simulink library "lib_IC_GFL"  (R2026a)
settings: Solver=VariableStepAuto
undefined symbols (not defined in the file): block_buses, block_DC_buses, block_DC_toM, block_idx, block_toM, buses_lf, DC, dparams, fref, invL, iTf, op_intconv_GFL, vdc_idx
libraries: sl_discontinuities x2, simulink x1
settings Model: Creator=atomas  LastModifiedBy=atomas

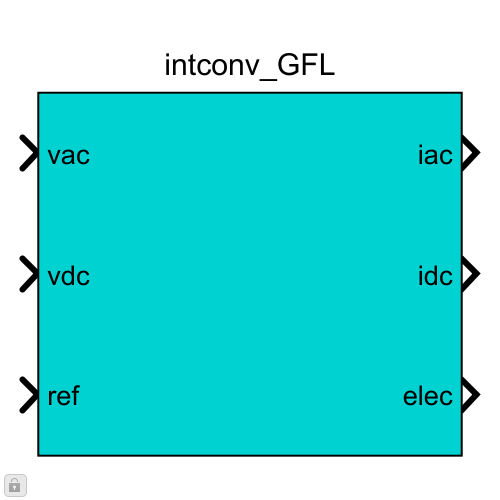
[thumbnail: Simulink's stored preview of the top-level diagram]
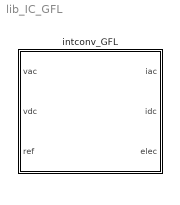
== system lib_IC_GFL ==
  intconv_GFL : Subsystem  mask(CCVSC){dynamic_CC=Dynamic, Tint=0.1, Kint=1, Bint=1, dynamic_PLL=Dynamic, kpi=1, kii=10, Tf=0.01, alphapcoef=0, alphaqcoef=0, Prel=1, Qrel=1, Eref=1, Kp_dc=0.5, Ki_dc=10}
      mask prompts: dynamic_CC "Dynamic behaviour"; dynamic_PLL "Dynamic behaviour"; Tf "LPF time constant (s)"; alphapcoef "P droop coefficient"; alphaqcoef "Q droop coefficient"; Prel "P/P_NmP"; Qrel "Q/Q_NnQ"; Eref "Nominal voltage of PCC"; Kp_dc "DC-voltage proportional gain Kp_dc (pu):"; Ki_dc "DC-voltage integral gain Ki_dc (pu/s):"
      mask help: Grid-following converter. CC is the current controller. Dynamic behavior includes the PI controller, decoupling and output inductance. Static behavior consists of setting the reference current directly in the output. PC is the power controller including the current reference calculation and low-pass filters for the power measurements.
      mask init:
      | [block_DC_buses, block_buses, block_DC_toM, block_toM, dparams, block_fref, block_idx, iTf, use_Tf, cc_mode, pll_mode, has_vdc_ctrl, vdc_idx] = mask_init_intconv_GFL(gcb, Tf, dynamic_CC, dynamic_PLL);
      mask Help: web('Documentation/CCVSC.html')
      mask TypeOptions dynamic_CC: Dynamic | Static
      mask TypeOptions dynamic_PLL: Dynamic | Static
      mask DialogControl CC Prompt: CC
      mask DialogControl PLL Prompt: PLL
      mask DialogControl PC Prompt: PC

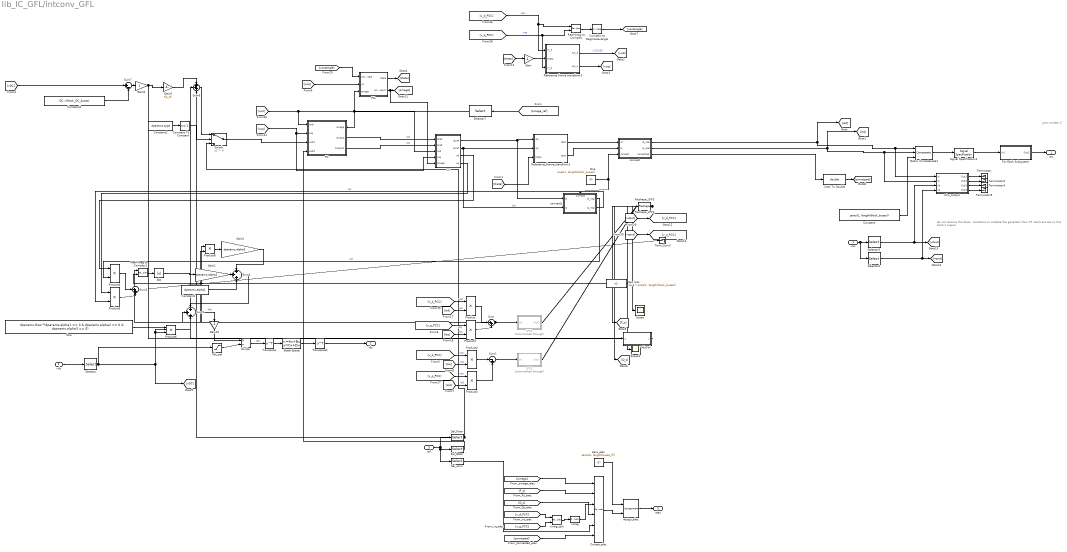
== system lib_IC_GFL/intconv_GFL ==
  note: port number 2
  note: do not rename this block, conditions to initialise the generator from PF result are set on this block's output
  vac : Inport
  vdc : Inport  Port=2
  ref : Inport  Port=3
  Abs : Abs  SaturateOnIntegerOverflow=off
  Assign_elec : Assignment  NumberOfDimensions=2  DiagnosticForDimensions=Warning  IndexOptions=Assign all,Index vector (dialog)  Indices=1,block_idx  OutputSizes=1
  CC : Subsystem  Variant=on
  Cast To Double : DataTypeConversion  OutDataTypeStr=double  SaturateOnIntegerOverflow=off  RndMeth=Floor
  Compare To Constant : simulink/Logic and Bit Operations/Compare To Constant  relop===  const=2  OutDataTypeStr=boolean
  Complex to Magnitude-Angle : ComplexToMagnitudeAngle  Output=Angle
  Concat_elec : Concatenate  NumInputs=6  Mode=Multidimensional array
  Constant : Constant  Value=zeros(1, length(block_buses))  VectorParams1D=off
  Constant1 : Constant  Value=dparams.alpha1  VectorParams1D=off
  Constant2 : Constant  Value=dparams.type  VectorParams1D=off
  Constant3 : Constant  Value=DC.v(block_DC_buses)  VectorParams1D=off
  Divide : Product  Inputs=*/
  Eps_loss : Constant  Value=1e-6 * ones(1, length(block_buses))  VectorParams1D=off
  For Each Subsystem : Subsystem  TreatAsAtomicUnit=on
  Gain : Gain  Gain=-1
  Gain1 : Gain  Gain=dparams.alpha2
  Gain10 : Gain  Gain=-1
  Gain2 : Gain  Gain=dparams.alpha3
  Gain5 : Gain  Gain=Kp_dc
  Gain9 : Gain
  Gsw : Constant  Value=dparams.Gsw.*(dparams.alpha1 == 0 & dparams.alpha2 == 0 & dparams.alpha3 == 0)  VectorParams1D=off
  LPF2 : Subsystem  Commented=through  Variant=on
  LPF3 : Subsystem  Commented=through  Variant=on
  Matrix Concatenate1 : Concatenate  NumInputs=3  Mode=Multidimensional array
  One : Constant  Value=ones(1, length(block_buses))  VectorParams1D=off  OutDataTypeStr=Inherit: Inherit via back propagation
  PC : Subsystem
      settings: PortSchema="{\"entries\":[{\"content\":{\"sides\":[{\"content\":{\"connectorIds\":[\"In1\",\"In2\",\"In3\",\"In4\"]},\"type\":\"ConnectorPlacement.EquallySpacedRectSide\",\"uuid\":\"7748ce6f-2dcc-431c-b3ea-0be9c3088b1d\"},{\"content\":{\"connectorIds\":[\"In5\",\"Out1\",\"Out2\"],\"side\":\"RIGHT\"},\"type\":\"ConnectorPlacement.EquallySpacedRectSide\",\"uuid\":\"af86fd8d-043b-4d20-8ee8-e7a977d706a8\"},{\"content\":{\"side\":\"TOP\"},\"type\":\"ConnectorPlacement.EquallySpacedRectSide\",\"uuid\":\"807e0dc6-0d59-4ea5-9557-3ccfd29c2ad0\"}]},\"type\":\"ConnectorPlacement.EquallySpacedConnector\",\"uuid\":\"c7fe00c5-0a0a-4038-b7ac-e659fb2aa4a7\"}],\"packageUris\":[\"http://schema.mathworks.com/mf0/Connector/R2020b\"],\"version\":\"1.0\"}"
  PLL : Subsystem  Variant=on
  Product{,1..5,8} (7 alike) : Product
  Product6 : Product  Inputs=3
  Real-Imag to Complex : RealImagToComplex
  Real-Imag to Complex1 : RealImagToComplex
  Reference frame transform3 : Subsystem
  Reference_frame_transform1 : Subsystem
  Reshape_LPF2 : Reshape  OutputDimensionality=Row vector (2-D)
  Reshape_LPF3 : Reshape  OutputDimensionality=Row vector (2-D)
  Scope : Scope
      settings: ActiveDisplayYMinimum=-0.01179  ActiveDisplayYMaximum=0.0098
  Scope1 : Scope
      settings: ActiveDisplayYMinimum=-0.59827  ActiveDisplayYMaximum=0.48453  DataLoggingVariableName=ScopeData2
  Sel_Pstar : Selector  NumberOfDimensions=2  InputPortWidth=3  IndexOptions=Index vector (dialog),Index vector (dialog)  Indices=2,block_idx  OutputSizes=1
  Sel_Qstar : Selector  NumberOfDimensions=2  InputPortWidth=3  IndexOptions=Index vector (dialog),Index vector (dialog)  Indices=4,block_idx  OutputSizes=1
  Sel_conn : Selector  NumberOfDimensions=2  InputPortWidth=3  IndexOptions=Index vector (dialog),Index vector (dialog)  Indices=5,block_idx  OutputSizes=1
  Selector : Selector  InputPortWidth=DC.Nbuses  IndexOptions=Index vector (dialog)  Indices=block_DC_buses  OutputSizes=1
  Selector5 : Selector  NumberOfDimensions=2  InputPortWidth=3  IndexOptions=Index vector (dialog),Index vector (dialog)  Indices=1,block_buses  OutputSizes=1,1
  Selector6 : Selector  NumberOfDimensions=2  InputPortWidth=3  IndexOptions=Index vector (dialog),Index vector (dialog)  Indices=2,block_buses  OutputSizes=1,1
  Selector7 : Selector  InputPortWidth=length(fref.ref_units)  IndexOptions=Index vector (dialog)  Indices=block_fref  OutputSizes=1
  Signal Specification1 : SignalSpecification  Dimensions=[3 length(block_buses)]
  State-Space : StateSpace  A=[]  B=[]  C=[]  D=block_DC_toM  InitialCondition=0  ParameterTunability=Optimized
  Sum : Sum  Inputs=|++
  Sum1 : Sum  Inputs=|-+
  Sum2 : Sum  Inputs=|++
  Sum4 : Sum  Inputs=+|+|+
  Sum5 : Sum  Inputs=+|+|+
  Sum6 : Sum  Inputs=+++
  Sum7 : Sum  Inputs=|+-
  Switch : Switch  Criteria=u2 > Threshold  SaturateOnIntegerOverflow=off  InputSameDT=off
  Term_Sum2 : Terminator
  Terminator{,3..5} (4 alike) : Terminator
  Transpose : Math  Operator=transpose
  Transpose1 : Math  Operator=transpose
  VdcCtrl : Subsystem  Variant=on
  Vdc_sat : Saturate  UpperLimit=inf  LowerLimit=0.1
  Zero_elec : Constant  Value=zeros(6, length(buses_lf))
  connect : Subsystem
  connect1 : Subsystem
      settings: PortSchema="{\"entries\":[{\"content\":{\"sides\":[{\"content\":{\"connectorIds\":[\"In1\",\"In2\"]},\"type\":\"ConnectorPlacement.EquallySpacedRectSide\",\"uuid\":\"6197940c-2174-4524-96b1-99ee20c84056\"},{\"content\":{\"connectorIds\":[\"Out1\",\"Out2\"],\"side\":\"RIGHT\"},\"type\":\"ConnectorPlacement.EquallySpacedRectSide\",\"uuid\":\"9096a550-ff71-4818-a7e7-327a4860b088\"},{\"content\":{\"connectorIds\":[\"In3\"],\"side\":\"TOP\"},\"type\":\"ConnectorPlacement.EquallySpacedRectSide\",\"uuid\":\"d804310e-982f-4fb4-ab62-6be4f27f3ef7\"}]},\"type\":\"ConnectorPlacement.EquallySpacedConnector\",\"uuid\":\"3c08874d-8366-4035-b771-5fa3fbbe507b\"}],\"packageUris\":[\"http://schema.mathworks.com/mf0/Connector/R2020b\"],\"version\":\"1.0\"}"
  trim_output : Subsystem
  vmag : ComplexToMagnitudeAngle  Output=Magnitude
  vmag_cplx : RealImagToComplex
  iac : Outport
  idc : Outport  Port=2
  elec : Outport  Port=3
  wires:
  Sum1/1 -> LPF3/1(In1)
  Sum/1 -> LPF2/1(In1), Sum5/2, Product8/1, Product8/2, Real-Imag to Complex1/1
  vac/1 -> Selector5/1, Selector6/1
  Selector6/1 -> [vqout], trim_output/4(vq)
  Selector5/1 -> [vdout], trim_output/3(vd)
  trim_output/4(Out4) -> Terminator5/1
  trim_output/2(Out2) -> Terminator3/1
  trim_output/3(Out3) -> Terminator4/1
  trim_output/1(Out1) -> Terminator/1
  For Each Subsystem/1(Out1) -> iac/1
  Constant/1 -> Matrix Concatenate1/3
  Signal Specification1/1 -> For Each Subsystem/1(In1)
  Matrix Concatenate1/1 -> Signal Specification1/1
  [v_q_PCC] -> Reference frame transform3/3(in_q), Real-Imag to Complex/2  "voq"
  [v_d_PCC] -> Reference frame transform3/1(in_d), Real-Imag to Complex/1  "vod"
  connect/2(iq_real) -> Matrix Concatenate1/2, trim_output/2(iq), [ioq]
  connect/1(id_real) -> Matrix Concatenate1/1, trim_output/1(id), [iod]
  One/1 -> connect/3(connect), connect1/3(connect)
  Cast To Double/1 -> [connected]
  Reference_frame_transform1/1(dout) -> connect/1(id)
  Reference_frame_transform1/2(qout) -> connect/2(iq)
  PLL/2(omega_point) -> [omega], CC/5(omega)
  Complex to Magnitude-Angle/1 -> [voutangle]
  Real-Imag to Complex/1 -> Complex to Magnitude-Angle/1
  [vod] -> CC/3(vod), PC/1(vodi)
  [voq] -> CC/4(voq), PC/2(voq)
  Reference frame transform3/1(out_d) -> [vod]  "v CCVSC"
  [v_q_PCC] -> Product1/1  "voq"
  [iod] -> Product3/2  "iod"
  [ioq] -> Product2/2  "ioq"
  Product2/1 -> Sum1/1
  Product1/1 -> Sum/2
  Product3/1 -> Sum1/2
  Product/1 -> Sum/1
  [v_d_PCC] -> Product/1  "vod"
  [iod] -> Product/2  "iod"
  [ioq] -> Product1/2  "ioq"
  [v_d_PCC] -> Product2/1  "vod"
  [v_q_PCC] -> Product3/1  "voq"
  PC/1(Output) -> CC/1(idref)  "iod"
  PC/2(Output1) -> CC/2(iqref)  "ioq"
  [theta] -> Gain/1
  Gain/1 -> Reference frame transform3/2(theta)
  [theta] -> Reference_frame_transform1/3(theta)
  [voq] -> PLL/2(vq)
  [omega_ref] -> Selector7/1
  PLL/1(theta) -> [theta]
  Reference frame transform3/2(out_q) -> [voq]
  connect/3(connected) -> Cast To Double/1
  [voutangle] -> PLL/1(voutangle)
  Product4/1 -> Sum2/1
  Product5/1 -> Sum2/2
  connect1/2(iq_real) -> Product5/2  "ioq"
  connect1/1(id_real) -> Product4/2  "iod"
  CC/3(vid) -> Product4/1
  CC/4(viq) -> Product5/1
  Real-Imag to Complex1/1 -> Abs/1
  Constant1/1 -> Sum4/3
  Gain1/1 -> Sum4/2
  Product8/1 -> Gain2/1
  Gain2/1 -> Sum4/1
  Sum5/1 -> Gain10/1  "Pdc"
  Divide/1 -> Transpose/1  "iDC"
  [vdout] -> [v_d_PCC]
  [vqout] -> [v_q_PCC]
  Switch/1 -> PC/3(vodi1)
  Constant2/1 -> Compare To Constant/1
  Gain5/1 -> Sum6/1
  Sum6/1 -> Switch/1
  Constant3/1 -> Sum7/2
  Gain9/1 -> Gain5/1, VdcCtrl/1(u)
  CC/1(idiref) -> connect1/1(id), Reference_frame_transform1/1(din)
  CC/2(iqiref) -> Reference_frame_transform1/2(qin), connect1/2(iq)  "ioq"
  Sum7/1 -> Gain9/1
  Compare To Constant/1 -> Switch/2
  Gain10/1 -> Divide/1
  Product6/1 -> Sum5/3
  Abs/1 -> Gain1/1
  Sum4/1 -> Sum5/1
  Gsw/1 -> Product6/1
  State-Space/1 -> Transpose1/1
  Transpose/1 -> State-Space/1
  [vDC] -> Sum7/1
  Selector7/1 -> PC/5(omega), PLL/3(omega)
  Transpose1/1 -> idc/1
  Selector/1 -> Product6/3, Product6/2, [vDC], Vdc_sat/1
  vdc/1 -> Selector/1
  ref/1 -> Sel_Qstar/1, Sel_conn/1, Sel_Pstar/1
  Sel_Pstar/1 -> Switch/3, Sum6/3
  Sel_Qstar/1 -> PC/4(vodi2)
  [v_d_PCC] -> vmag_cplx/1
  [v_q_PCC] -> vmag_cplx/2
  vmag_cplx/1 -> vmag/1
  [omega] -> Concat_elec/1
  [P_s] -> Concat_elec/2
  vmag/1 -> Concat_elec/3
  [Q_s] -> Concat_elec/4
  Sel_conn/1 -> Concat_elec/5
  [connected] -> Concat_elec/6
  Zero_elec/1 -> Assign_elec/1
  Concat_elec/1 -> Assign_elec/2
  Assign_elec/1 -> elec/1
  Vdc_sat/1 -> Divide/2
  VdcCtrl/1(y) -> Sum6/2
  Sum2/1 -> Term_Sum2/1
  Eps_loss/1 -> Real-Imag to Complex1/2
  LPF2/1(Out1) -> Reshape_LPF2/1
  Reshape_LPF2/1 -> Scope/1, [P_s]
  LPF3/1(Out1) -> Reshape_LPF3/1
  Reshape_LPF3/1 -> Scope1/1, [Q_s]

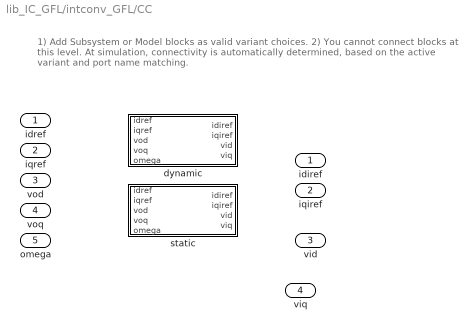
== system lib_IC_GFL/intconv_GFL/CC ==
  note: 1) Add Subsystem or Model blocks as valid variant choices.
      | 2) You cannot connect blocks at this level. At simulation, connectivity is automatically
      | determined, based on the active variant and port name matching.
  idref : Inport
  iqref : Inport  Port=2
  vod : Inport  Port=3
  voq : Inport  Port=4
  omega : Inport  Port=5
  dynamic : Subsystem  VariantControl=cc_mode == 1  mask{dynamic_line=Dynamic}
      mask prompts: dynamic_line "Line"
      mask TypeOptions dynamic_line: RL/dynamic
  static : Subsystem  VariantControl=(default)
  idiref : Outport
  iqiref : Outport  Port=2
  vid : Outport  Port=3
  viq : Outport  Port=4

== system lib_IC_GFL/intconv_GFL/For Each Subsystem ==
  In1 : Inport  Partition=on  PartitionDimension=1  PartitionWidth=1  PartitionOffset=0
  For Each : ForEach  DisableCoverage=on
  State-Space : StateSpace  A=[]  B=[]  C=[]  D=block_toM  InitialCondition=0  ParameterTunability=Optimized
  Transpose : Math  Operator=transpose
  Transpose1 : Math  Operator=transpose
  Out1 : Outport  ConcatenationDimension=1
  wires:
  In1/1 -> Transpose/1
  Transpose1/1 -> Out1/1
  Transpose/1 -> State-Space/1
  State-Space/1 -> Transpose1/1

== system lib_IC_GFL/intconv_GFL/LPF2 ==
  note: 1) Add Subsystem or Model blocks as valid variant choices.
      | 2) You cannot connect blocks at this level. At simulation, connectivity is automatically
      | determined, based on the active variant and port name matching.
  In1 : Inport
  Active : Subsystem  VariantControl=use_Tf == 1
  Bypass : Subsystem  VariantControl=(default)
  Out1 : Outport

== system lib_IC_GFL/intconv_GFL/LPF3 ==
  note: 1) Add Subsystem or Model blocks as valid variant choices.
      | 2) You cannot connect blocks at this level. At simulation, connectivity is automatically
      | determined, based on the active variant and port name matching.
  In1 : Inport
  Active : Subsystem  VariantControl=use_Tf == 1
  Bypass : Subsystem  VariantControl=(default)
  Out1 : Outport

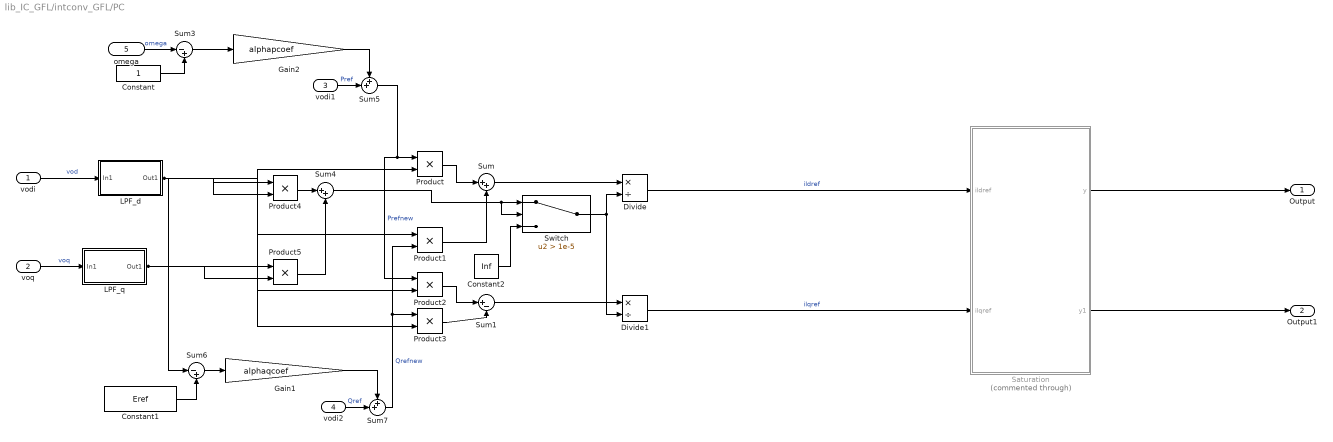
== system lib_IC_GFL/intconv_GFL/PC ==
  vodi : Inport
  voq : Inport  Port=2
  vodi1 : Inport  Port=3
  vodi2 : Inport  Port=4
  omega : Inport  Port=5
  Constant : Constant
  Constant1 : Constant  Value=Eref  VectorParams1D=off
  Constant2 : Constant  Value=Inf
  Divide : Product  Inputs=*/
  Divide1 : Product  Inputs=*/
  Gain1 : Gain  Gain=alphaqcoef
  Gain2 : Gain  Gain=alphapcoef
  LPF_d : Subsystem  Variant=on
  LPF_q : Subsystem  Variant=on
  Product{,1..5} (6 alike) : Product
  Saturation : Subsystem  Commented=through
  Sum : Sum  Inputs=|++
  Sum1 : Sum  Inputs=|+-
  Sum3 : Sum  Inputs=|-+
  Sum4 : Sum  Inputs=|++
  Sum5 : Sum  Inputs=++|
  Sum6 : Sum  Inputs=|-+
  Sum7 : Sum  Inputs=++|
  Switch : Switch  Criteria=u2 > Threshold  Threshold=1e-5  ZeroCross=off  SaturateOnIntegerOverflow=off  InputSameDT=off
  Output : Outport
  Output1 : Outport  Port=2
  wires:
  LPF_q/1(Out1) -> Product1/1, Product2/2, Product5/2, Product5/1
  voq/1 -> LPF_q/1(In1)  "voq"
  LPF_d/1(Out1) -> Sum6/1, Product3/2, Product/2, Product4/2, Product4/1
  vodi/1 -> LPF_d/1(In1)  "vod"
  Saturation/2(y1) -> Output1/1
  Saturation/1(y) -> Output/1
  Divide1/1 -> Saturation/2(ilqref)  "ilqref"
  Divide/1 -> Saturation/1(ildref)  "ildref"
  Product/1 -> Sum/1
  Product1/1 -> Sum/2
  Product2/1 -> Sum1/1
  Product3/1 -> Sum1/2
  Sum7/1 -> Product1/2, Product3/1  "Qrefnew"
  Product4/1 -> Sum4/1
  Product5/1 -> Sum4/2
  Sum5/1 -> Product2/1, Product/1  "Prefnew"
  Sum1/1 -> Divide1/1
  Sum4/1 -> Switch/2, Switch/1
  Sum/1 -> Divide/1
  Sum3/1 -> Gain2/1
  Constant/1 -> Sum3/2
  Gain2/1 -> Sum5/1
  vodi1/1 -> Sum5/2  "Pref"
  Constant1/1 -> Sum6/2
  Gain1/1 -> Sum7/1
  omega/1 -> Sum3/1  "omega"
  Sum6/1 -> Gain1/1
  vodi2/1 -> Sum7/2  "Qref"
  Constant2/1 -> Switch/3
  Switch/1 -> Divide/2, Divide1/2

== system lib_IC_GFL/intconv_GFL/PLL ==
  note: 1) Add Subsystem or Model blocks as valid variant choices.
      | 2) You cannot connect blocks at this level. At simulation, connectivity is automatically
      | determined, based on the active variant and port name matching.
  voutangle : Inport
  vq : Inport  Port=2
  omega : Inport  Port=3
  dynamic : Subsystem  VariantControl=pll_mode == 1
  static : Subsystem  VariantControl=(default)
  theta : Outport
  omega_point : Outport  Port=2

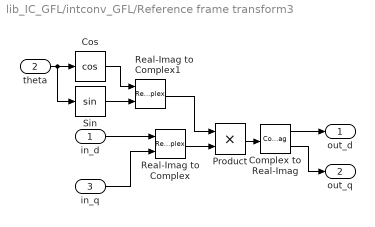
== system lib_IC_GFL/intconv_GFL/Reference frame transform3 ==
  in_d : Inport
  theta : Inport  Port=2
  in_q : Inport  Port=3
  Complex to Real-Imag : ComplexToRealImag
  Cos : Trigonometry  SCDEnableBlockLinearizationSpecification=on  Operator=cos
  Product : Product
  Real-Imag to Complex : RealImagToComplex
  Real-Imag to Complex1 : RealImagToComplex
  Sin : Trigonometry  SCDEnableBlockLinearizationSpecification=on
  out_d : Outport
  out_q : Outport  Port=2
  wires:
  in_d/1 -> Real-Imag to Complex/1
  in_q/1 -> Real-Imag to Complex/2
  Complex to Real-Imag/1 -> out_d/1
  Sin/1 -> Real-Imag to Complex1/2
  Cos/1 -> Real-Imag to Complex1/1
  theta/1 -> Cos/1, Sin/1
  Product/1 -> Complex to Real-Imag/1
  Real-Imag to Complex/1 -> Product/2
  Real-Imag to Complex1/1 -> Product/1
  Complex to Real-Imag/2 -> out_q/1

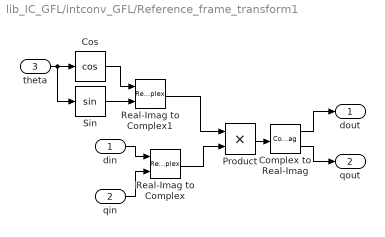
== system lib_IC_GFL/intconv_GFL/Reference_frame_transform1 ==
  din : Inport
  qin : Inport  Port=2
  theta : Inport  Port=3
  Complex to Real-Imag : ComplexToRealImag
  Cos : Trigonometry  SCDEnableBlockLinearizationSpecification=on  Operator=cos
  Product : Product
  Real-Imag to Complex : RealImagToComplex
  Real-Imag to Complex1 : RealImagToComplex
  Sin : Trigonometry  SCDEnableBlockLinearizationSpecification=on
  dout : Outport
  qout : Outport  Port=2
  wires:
  Complex to Real-Imag/1 -> dout/1
  Complex to Real-Imag/2 -> qout/1
  Real-Imag to Complex1/1 -> Product/1
  din/1 -> Real-Imag to Complex/1
  qin/1 -> Real-Imag to Complex/2
  Real-Imag to Complex/1 -> Product/2
  Product/1 -> Complex to Real-Imag/1
  theta/1 -> Sin/1, Cos/1
  Cos/1 -> Real-Imag to Complex1/1
  Sin/1 -> Real-Imag to Complex1/2

== system lib_IC_GFL/intconv_GFL/VdcCtrl ==
  note: 1) Add Subsystem or Model blocks as valid variant choices.
      | 2) You cannot connect blocks at this level. At simulation, connectivity is automatically
      | determined, based on the active variant and port name matching.
  u : Inport
  Active : Subsystem  VariantControl=has_vdc_ctrl == 1
  Bypass : Subsystem  VariantControl=(default)
  y : Outport

== system lib_IC_GFL/intconv_GFL/connect ==
  id : Inport
  iq : Inport  Port=2
  connect : Inport  Port=3
  Switch : Switch  Criteria=u2 > Threshold  ZeroCross=off  SaturateOnIntegerOverflow=off  InputSameDT=off
  Switch1 : Switch  Criteria=u2 > Threshold  ZeroCross=off  SaturateOnIntegerOverflow=off  InputSameDT=off
  Zero1 : Constant  Value=0  VectorParams1D=off  OutDataTypeStr=Inherit: Inherit via back propagation
  Zero2 : Constant  Value=0  VectorParams1D=off  OutDataTypeStr=Inherit: Inherit via back propagation
  id_real : Outport
  iq_real : Outport  Port=2
  connected : Outport  Port=3  OutDataTypeStr=boolean
  wires:
  Zero2/1 -> Switch1/3
  iq/1 -> Switch1/1
  Switch1/1 -> iq_real/1
  connect/1 -> Switch/2, Switch1/2, connected/1
  id/1 -> Switch/1
  Zero1/1 -> Switch/3
  Switch/1 -> id_real/1

== system lib_IC_GFL/intconv_GFL/connect1 ==
  id : Inport
  iq : Inport  Port=2
  connect : Inport  Port=3
  Switch : Switch  Criteria=u2 > Threshold  ZeroCross=off  SaturateOnIntegerOverflow=off  InputSameDT=off
  Switch1 : Switch  Criteria=u2 > Threshold  ZeroCross=off  SaturateOnIntegerOverflow=off  InputSameDT=off
  Zero1 : Constant  Value=0  VectorParams1D=off  OutDataTypeStr=Inherit: Inherit via back propagation
  Zero2 : Constant  Value=0  VectorParams1D=off  OutDataTypeStr=Inherit: Inherit via back propagation
  id_real : Outport
  iq_real : Outport  Port=2
  wires:
  Switch/1 -> id_real/1
  Zero1/1 -> Switch/3
  id/1 -> Switch/1
  connect/1 -> Switch1/2, Switch/2
  Switch1/1 -> iq_real/1
  iq/1 -> Switch1/1
  Zero2/1 -> Switch1/3

== system lib_IC_GFL/intconv_GFL/trim_output ==
  id : Inport
  iq : Inport  Port=2
  vd : Inport  Port=3
  vq : Inport  Port=4
  Out1 : Outport
  Out2 : Outport  Port=2
  Out3 : Outport  Port=3
  Out4 : Outport  Port=4
  wires:
  iq/1 -> Out2/1
  vd/1 -> Out3/1
  vq/1 -> Out4/1
  id/1 -> Out1/1

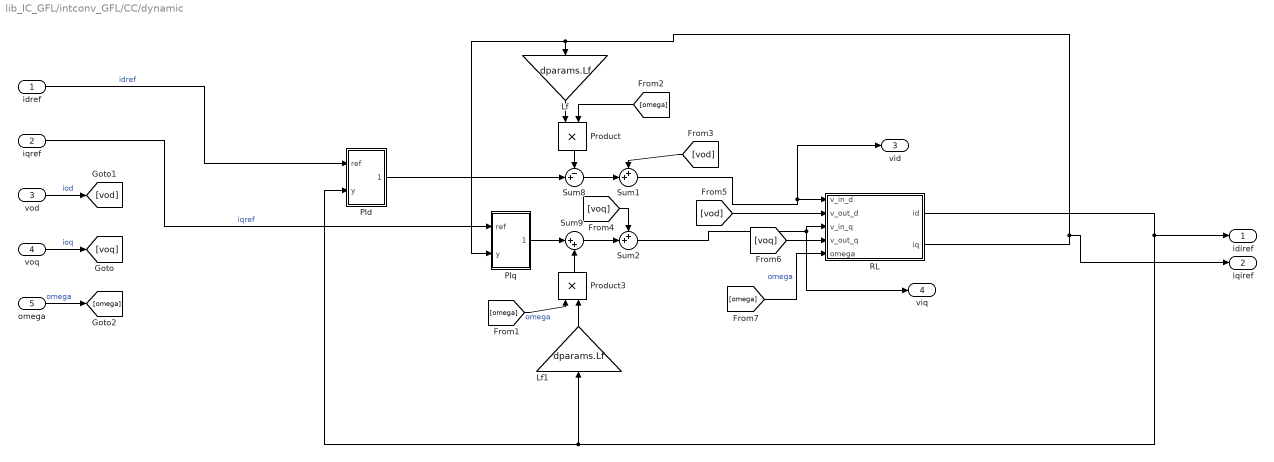
== system lib_IC_GFL/intconv_GFL/CC/dynamic ==
  idref : Inport
  iqref : Inport  Port=2
  vod : Inport  Port=3
  voq : Inport  Port=4
  omega : Inport  Port=5
  "Lf " : Gain  Gain=dparams.Lf
  Lf1 : Gain  Gain=dparams.Lf
  PId : Subsystem
  PIq : Subsystem
  Product : Product
  Product3 : Product
  RL : Subsystem  Variant=on  mask(Line){dynamic=Dynamic, R=dparams.Rf, L=dparams.Lf}
      mask prompts: dynamic "Dynamic behavior"; R "Series resistance (p.u.)"; L "Inductance (p.u.)"
      mask init:
      | [invL, omegab, rl_mode] = mask_init_RL(dynamic, L, 50);
      mask Help: web('Documentation/RL.html')
      mask TypeOptions dynamic: Static | Dynamic | Static omega
  Sum1 : Sum  Inputs=++|
  Sum2 : Sum  Inputs=++|
  Sum8 : Sum  Inputs=-+|
  Sum9 : Sum  Inputs=|++
  idiref : Outport
  iqiref : Outport  Port=2
  vid : Outport  Port=3
  viq : Outport  Port=4
  wires:
  PId/1(Out1) -> Sum8/2
  idref/1 -> PId/1(ref)  "idref"
  RL/1(id) -> idiref/1, Lf1/1, PId/2(y)
  Sum2/1 -> viq/1, RL/3(v_in_q)
  Sum1/1 -> vid/1, RL/1(v_in_d)
  [voq] -> RL/4(v_out_q)
  [vod] -> RL/2(v_out_d)
  vod/1 -> [vod]  "iod"
  voq/1 -> [voq]  "ioq"
  omega/1 -> [omega]  "omega"
  [voq] -> Sum2/1
  [vod] -> Sum1/1
  Sum9/1 -> Sum2/2
  Sum8/1 -> Sum1/2
  iqref/1 -> PIq/1(ref)  "iqref"
  Product/1 -> Sum8/1
  [omega] -> Product/2
  Lf1/1 -> Product3/2
  Product3/1 -> Sum9/2
  "Lf "/1 -> Product/1
  [omega] -> Product3/1  "omega"
  PIq/1(Out1) -> Sum9/1
  RL/2(iq) -> "Lf "/1, PIq/2(y), iqiref/1
  [omega] -> RL/5(omega)  "omega"

== system lib_IC_GFL/intconv_GFL/CC/static ==
  idref : Inport
  iqref : Inport  Port=2
  vod : Inport  Port=3
  voq : Inport  Port=4
  omega : Inport  Port=5
  Terminator2 : Terminator
  idiref : Outport
  iqiref : Outport  Port=2
  vid : Outport  Port=3
  viq : Outport  Port=4
  wires:
  omega/1 -> Terminator2/1  "omega"
  iqref/1 -> iqiref/1  "iqref"
  idref/1 -> idiref/1  "idref"
  vod/1 -> vid/1  "vod"
  voq/1 -> viq/1  "voq"

== system lib_IC_GFL/intconv_GFL/LPF2/Active ==
  In1 : Inport
  Impl : Subsystem
  Out1 : Outport
  wires:
  Impl/1(Out1) -> Out1/1
  In1/1 -> Impl/1(In1)

== system lib_IC_GFL/intconv_GFL/LPF2/Bypass ==
  In1 : Inport
  Reshape_row : Reshape  OutputDimensionality=Row vector (2-D)
  Out1 : Outport
  wires:
  In1/1 -> Reshape_row/1
  Reshape_row/1 -> Out1/1

== system lib_IC_GFL/intconv_GFL/LPF3/Active ==
  In1 : Inport
  Impl : Subsystem
  Out1 : Outport
  wires:
  Impl/1(Out1) -> Out1/1
  In1/1 -> Impl/1(In1)

== system lib_IC_GFL/intconv_GFL/LPF3/Bypass ==
  In1 : Inport
  Reshape_row : Reshape  OutputDimensionality=Row vector (2-D)
  Out1 : Outport
  wires:
  In1/1 -> Reshape_row/1
  Reshape_row/1 -> Out1/1

== system lib_IC_GFL/intconv_GFL/PC/LPF_d ==
  note: 1) Add Subsystem or Model blocks as valid variant choices.
      | 2) You cannot connect blocks at this level. At simulation, connectivity is automatically
      | determined, based on the active variant and port name matching.
  In1 : Inport
  Active : Subsystem  VariantControl=use_Tf == 1
  Bypass : Subsystem  VariantControl=(default)
  Out1 : Outport

== system lib_IC_GFL/intconv_GFL/PC/LPF_q ==
  note: 1) Add Subsystem or Model blocks as valid variant choices.
      | 2) You cannot connect blocks at this level. At simulation, connectivity is automatically
      | determined, based on the active variant and port name matching.
  In1 : Inport
  Active : Subsystem  VariantControl=use_Tf == 1
  Bypass : Subsystem  VariantControl=(default)
  Out1 : Outport

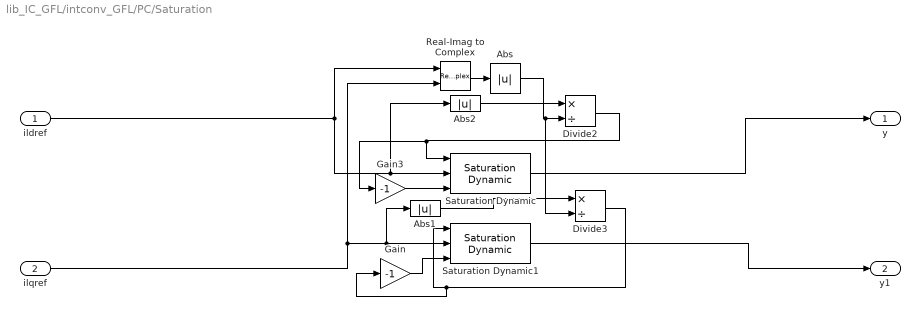
== system lib_IC_GFL/intconv_GFL/PC/Saturation ==
  ildref : Inport
  ilqref : Inport  Port=2
  Abs : Abs  ZeroCross=off  SaturateOnIntegerOverflow=off
  Abs1 : Abs  ZeroCross=off  SaturateOnIntegerOverflow=off
  Abs2 : Abs  ZeroCross=off  SaturateOnIntegerOverflow=off
  Divide2 : Product  Inputs=*/
  Divide3 : Product  Inputs=*/
  Gain : Gain  Gain=-1
  Gain3 : Gain  Gain=-1
  Real-Imag to Complex : RealImagToComplex
  Saturation Dynamic : sl_discontinuities/Saturation Dynamic  OutMin=[]  OutMax=[]  OutDataTypeStr=Inherit: Same as second input  OutDataType=fixdt(1, 16)  OutScaling=2^-10  DoSatur=off
  Saturation Dynamic1 : sl_discontinuities/Saturation Dynamic  OutMin=[]  OutMax=[]  OutDataTypeStr=Inherit: Same as second input  OutDataType=fixdt(1, 16)  OutScaling=2^-10  DoSatur=off
  y : Outport
  y1 : Outport  Port=2
  wires:
  Saturation Dynamic1/1 -> y1/1
  ildref/1 -> Real-Imag to Complex/1, Saturation Dynamic/2, Abs2/1
  Abs2/1 -> Divide2/1
  ilqref/1 -> Real-Imag to Complex/2, Saturation Dynamic1/2, Abs1/1
  Real-Imag to Complex/1 -> Abs/1
  Abs1/1 -> Divide3/1
  Gain3/1 -> Saturation Dynamic/3
  Abs/1 -> Divide2/2, Divide3/2
  Saturation Dynamic/1 -> y/1
  Divide2/1 -> Saturation Dynamic/1, Gain3/1
  Divide3/1 -> Saturation Dynamic1/1, Gain/1
  Gain/1 -> Saturation Dynamic1/3

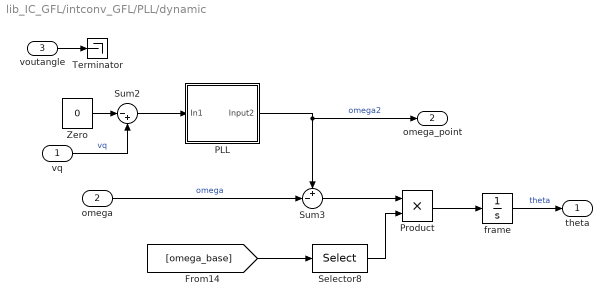
== system lib_IC_GFL/intconv_GFL/PLL/dynamic ==
  vq : Inport
  omega : Inport  Port=2
  voutangle : Inport  Port=3
  PLL : Subsystem
  Product : Product
  Selector8 : Selector  InputPortWidth=length(fref.ref_units)  IndexOptions=Index vector (dialog)  Indices=block_fref  OutputSizes=1
  Sum2 : Sum  Inputs=|-+
  Sum3 : Sum  Inputs=+-|
  Terminator : Terminator
  Zero : Constant  Value=0  OutDataTypeStr=Inherit: Inherit via back propagation
  frame : Integrator  InitialCondition=op_intconv_GFL.PLL_dynamic_frame  UpperSaturationLimit=pi  LowerSaturationLimit=-pi
  theta : Outport
  omega_point : Outport  Port=2
  wires:
  Sum2/1 -> PLL/1(In1)
  Sum3/1 -> Product/1
  PLL/1(Input2) -> Sum3/1, omega_point/1  "omega2"
  Product/1 -> frame/1
  frame/1 -> theta/1  "theta"
  Zero/1 -> Sum2/1
  omega/1 -> Sum3/2  "omega"
  vq/1 -> Sum2/2  "vq"
  voutangle/1 -> Terminator/1
  [omega_base] -> Selector8/1
  Selector8/1 -> Product/2

== system lib_IC_GFL/intconv_GFL/PLL/static ==
  vq : Inport
  omega : Inport  Port=2
  voutangle : Inport  Port=3
  Gain : Gain  Gain=-1
  IC : InitialCondition  Value=op_intconv_GFL.PLL_dynamic_frame
  Terminator : Terminator
  Terminator1 : Terminator
  theta : Outport
  omega_point : Outport  Port=2
  wires:
  voutangle/1 -> Gain/1
  omega/1 -> Terminator1/1, omega_point/1  "vq"
  vq/1 -> Terminator/1  "vq"
  Gain/1 -> IC/1
  IC/1 -> theta/1

== system lib_IC_GFL/intconv_GFL/VdcCtrl/Active ==
  u : Inport
  Asgn_vdc : Assignment  NumberOfDimensions=2  IndexOptions=Assign all,Index vector (dialog)  Indices=1,vdc_idx  OutputSizes=1
  Gain_Ki : Gain  Gain=reshape(Ki_dc(vdc_idx), 1, [])
  I : Integrator  InitialCondition=reshape(op_intconv_GFL.I, 1, [])
  Reshape_in : Reshape  OutputDimensionality=Row vector (2-D)
  Sel_vdc : Selector  NumberOfDimensions=2  IndexOptions=Select all,Index vector (dialog)  Indices=1,vdc_idx  OutputSizes=1
  Zero_vec : Constant  Value=zeros(1, length(block_buses))  VectorParams1D=off
  y : Outport
  wires:
  u/1 -> Reshape_in/1
  Reshape_in/1 -> Sel_vdc/1
  Sel_vdc/1 -> I/1
  I/1 -> Gain_Ki/1
  Zero_vec/1 -> Asgn_vdc/1
  Gain_Ki/1 -> Asgn_vdc/2
  Asgn_vdc/1 -> y/1

== system lib_IC_GFL/intconv_GFL/VdcCtrl/Bypass ==
  u : Inport
  Term : Terminator
  Zero_vec : Constant  Value=zeros(1, length(block_buses))  VectorParams1D=off
  y : Outport
  wires:
  u/1 -> Term/1
  Zero_vec/1 -> y/1

== system lib_IC_GFL/intconv_GFL/CC/dynamic/PId ==
  ref : Inport
  y : Inport  Port=2
  Gain : Gain  Gain=Bint
  Gain1 : Gain  Gain=1./Tint
  Gain2 : Gain  Gain=Kint
  I : Integrator  InitialCondition=op_intconv_GFL.CC_dynamic_PId_I
  Sum : Sum  Inputs=++|
  Sum1 : Sum  Inputs=|+-
  Sum6 : Sum  Inputs=|+-
  Out1 : Outport
  wires:
  Gain2/1 -> Out1/1
  I/1 -> Sum/2
  Gain1/1 -> I/1
  Sum6/1 -> Gain1/1
  Sum1/1 -> Sum/1
  Sum/1 -> Gain2/1
  Gain/1 -> Sum1/1
  ref/1 -> Sum6/1, Gain/1
  y/1 -> Sum6/2, Sum1/2

== system lib_IC_GFL/intconv_GFL/CC/dynamic/PIq ==
  ref : Inport
  y : Inport  Port=2
  Gain : Gain  Gain=Bint
  Gain1 : Gain  Gain=1./Tint
  Gain2 : Gain  Gain=Kint
  I : Integrator  InitialCondition=op_intconv_GFL.CC_dynamic_PIq_I
  Sum : Sum  Inputs=++|
  Sum1 : Sum  Inputs=|+-
  Sum6 : Sum  Inputs=|+-
  Out1 : Outport
  wires:
  y/1 -> Sum1/2, Sum6/2
  ref/1 -> Gain/1, Sum6/1
  Gain/1 -> Sum1/1
  Sum/1 -> Gain2/1
  Sum1/1 -> Sum/1
  Sum6/1 -> Gain1/1
  Gain1/1 -> I/1
  I/1 -> Sum/2
  Gain2/1 -> Out1/1

== system lib_IC_GFL/intconv_GFL/CC/dynamic/RL ==
  note: 1) Add Subsystem or Model blocks as valid variant choices.
      | 2) You cannot connect blocks at this level. At simulation, connectivity is automatically
      | determined, based on the active variant and port name matching.
  v_in_d : Inport
  v_out_d : Inport  Port=2
  v_in_q : Inport  Port=3
  v_out_q : Inport  Port=4
  omega : Inport  Port=5
  dynamic : Subsystem  VariantControl=rl_mode == 1
      settings: PortSchema="{\"entries\":[{\"content\":{\"sides\":[{\"content\":{\"connectorIds\":[\"In1\"]},\"type\":\"ConnectorPlacement.EquallySpacedRectSide\",\"uuid\":\"63966e24-f9e7-4b2d-b456-7f4ea5e3f230\"},{\"content\":{\"connectorIds\":[\"In2\",\"In3\",\"In4\",\"In5\",\"Out1\",\"Out2\"],\"side\":\"RIGHT\"},\"type\":\"ConnectorPlacement.EquallySpacedRectSide\",\"uuid\":\"ded6ef04-52fd-47df-8e49-cf16b827098d\"},{\"content\":{\"side\":\"TOP\"},\"type\":\"ConnectorPlacement.EquallySpacedRectSide\",\"uuid\":\"f940a985-fa23-4968-ad44-1d76d0e20c6a\"}]},\"type\":\"ConnectorPlacement.EquallySpacedConnector\",\"uuid\":\"20f61d3c-9af2-4982-98ea-af4910e61c9c\"}],\"packageUris\":[\"http://schema.mathworks.com/mf0/Connector/R2020b\"],\"version\":\"1.0\"}"
  static : Subsystem  VariantControl=rl_mode == 2
  static_omega : Subsystem  VariantControl=(default)
  id : Outport
  iq : Outport  Port=2

== system lib_IC_GFL/intconv_GFL/LPF2/Active/Impl ==
  In1 : Inport
  Gain : Gain  Gain=iTf
  I : Integrator  InitialCondition=op_intconv_GFL.LPF2_Active_Impl_I
  Sum4 : Sum  Inputs=|+-
  Out1 : Outport
  wires:
  I/1 -> Sum4/2, Out1/1
  In1/1 -> Sum4/1
  Sum4/1 -> Gain/1
  Gain/1 -> I/1

== system lib_IC_GFL/intconv_GFL/LPF3/Active/Impl ==
  In1 : Inport
  Gain : Gain  Gain=iTf
  I : Integrator  InitialCondition=op_intconv_GFL.LPF3_Active_Impl_I
  Sum4 : Sum  Inputs=|+-
  Out1 : Outport
  wires:
  Sum4/1 -> Gain/1
  In1/1 -> Sum4/1
  I/1 -> Sum4/2, Out1/1
  Gain/1 -> I/1

== system lib_IC_GFL/intconv_GFL/PC/LPF_d/Active ==
  In1 : Inport
  Impl : Subsystem
  Out1 : Outport
  wires:
  Impl/1(Out1) -> Out1/1
  In1/1 -> Impl/1(In1)

== system lib_IC_GFL/intconv_GFL/PC/LPF_d/Bypass ==
  In1 : Inport
  Out1 : Outport
  wires:
  In1/1 -> Out1/1

== system lib_IC_GFL/intconv_GFL/PC/LPF_q/Active ==
  In1 : Inport
  Impl : Subsystem
  Out1 : Outport
  wires:
  Impl/1(Out1) -> Out1/1
  In1/1 -> Impl/1(In1)

== system lib_IC_GFL/intconv_GFL/PC/LPF_q/Bypass ==
  In1 : Inport
  Out1 : Outport
  wires:
  In1/1 -> Out1/1

== system lib_IC_GFL/intconv_GFL/PLL/dynamic/PLL ==
  In1 : Inport
  Gain : Gain  Gain=kpi
  Gain1 : Gain  Gain=kii
  I : Integrator  InitialCondition=op_intconv_GFL.PLL_dynamic_PLL_I
  Sum10 : Sum  Inputs=|++
  Input2 : Outport
  wires:
  Sum10/1 -> Input2/1
  In1/1 -> Gain1/1, Gain/1
  Gain1/1 -> I/1
  Gain/1 -> Sum10/1
  I/1 -> Sum10/2

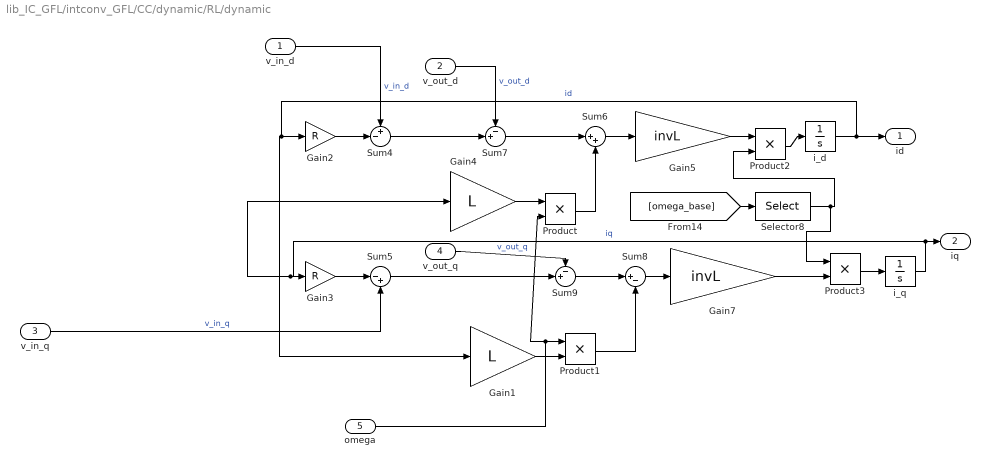
== system lib_IC_GFL/intconv_GFL/CC/dynamic/RL/dynamic ==
  v_in_d : Inport
  v_out_d : Inport  Port=2
  v_in_q : Inport  Port=3
  v_out_q : Inport  Port=4
  omega : Inport  Port=5
  Gain1 : Gain  Gain=L
  Gain2 : Gain  Gain=R
  Gain3 : Gain  Gain=R
  Gain4 : Gain  Gain=L
  Gain5 : Gain  Gain=invL
  Gain7 : Gain  Gain=invL
  Product{,1..3} (4 alike) : Product
  Selector8 : Selector  InputPortWidth=length(fref.ref_units)  IndexOptions=Index vector (dialog)  Indices=block_fref  OutputSizes=1
  Sum4 : Sum  Inputs=+-|
  Sum5 : Sum  Inputs=|-+
  Sum6 : Sum  Inputs=|++
  Sum7 : Sum  Inputs=-+|
  Sum8 : Sum  Inputs=|+-
  Sum9 : Sum  Inputs=-+|
  i_d : Integrator  InitialCondition=op_intconv_GFL.CC_dynamic_RL_dynamic_i_d
  i_q : Integrator  InitialCondition=op_intconv_GFL.CC_dynamic_RL_dynamic_i_q
  id : Outport
  iq : Outport  Port=2
  wires:
  v_in_q/1 -> Sum5/2  "v_in_q"
  v_in_d/1 -> Sum4/1  "v_in_d"
  Gain2/1 -> Sum4/2
  i_d/1 -> Gain2/1, Gain1/1, id/1  "id"
  Sum6/1 -> Gain5/1
  Product/1 -> Sum6/2
  Sum8/1 -> Gain7/1
  Sum4/1 -> Sum7/2
  Product1/1 -> Sum8/2
  Gain4/1 -> Product/1
  Sum7/1 -> Sum6/1
  Gain3/1 -> Sum5/1
  Sum5/1 -> Sum9/2
  i_q/1 -> Gain3/1, Gain4/1, iq/1  "iq"
  Gain1/1 -> Product1/2
  Sum9/1 -> Sum8/1
  v_out_d/1 -> Sum7/1  "v_out_d"
  v_out_q/1 -> Sum9/1  "v_out_q"
  omega/1 -> Product1/1, Product/2
  Gain5/1 -> Product2/1
  Product2/1 -> i_d/1
  Gain7/1 -> Product3/2
  Product3/1 -> i_q/1
  [omega_base] -> Selector8/1
  Selector8/1 -> Product3/1, Product2/2

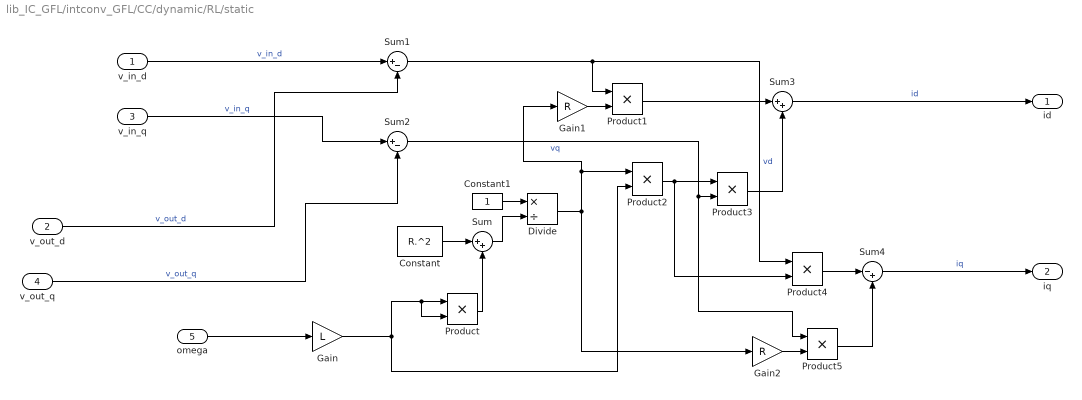
== system lib_IC_GFL/intconv_GFL/CC/dynamic/RL/static ==
  v_in_d : Inport
  v_out_d : Inport  Port=2
  v_in_q : Inport  Port=3
  v_out_q : Inport  Port=4
  omega : Inport  Port=5
  Constant : Constant  Value=R.^2
  Constant1 : Constant
  Divide : Product  Inputs=*/
  Gain : Gain  Gain=L
  Gain1 : Gain  Gain=R
  Gain2 : Gain  Gain=R
  Product{,1..5} (6 alike) : Product
  Sum : Sum  Inputs=|++
  Sum1 : Sum  Inputs=|+-
  Sum2 : Sum  Inputs=|+-
  Sum3 : Sum  Inputs=|++
  Sum4 : Sum  Inputs=|-+
  id : Outport
  iq : Outport  Port=2
  wires:
  v_in_q/1 -> Sum2/1  "v_in_q"
  v_out_d/1 -> Sum1/2  "v_out_d"
  Sum/1 -> Divide/2
  Gain2/1 -> Product5/2
  Product/1 -> Sum/2
  Product1/1 -> Sum3/1
  Product5/1 -> Sum4/2
  Constant/1 -> Sum/1
  Sum2/1 -> Product3/2, Product5/1  "vq"
  Gain/1 -> Product2/2, Product/1, Product/2
  Constant1/1 -> Divide/1
  Product3/1 -> Sum3/2
  Sum1/1 -> Product4/1, Product1/1  "vd"
  Divide/1 -> Product2/1, Gain1/1, Gain2/1
  Product4/1 -> Sum4/1
  Product2/1 -> Product3/1, Product4/2
  Gain1/1 -> Product1/2
  Sum3/1 -> id/1  "id"
  Sum4/1 -> iq/1  "iq"
  v_out_q/1 -> Sum2/2  "v_out_q"
  v_in_d/1 -> Sum1/1  "v_in_d"
  omega/1 -> Gain/1

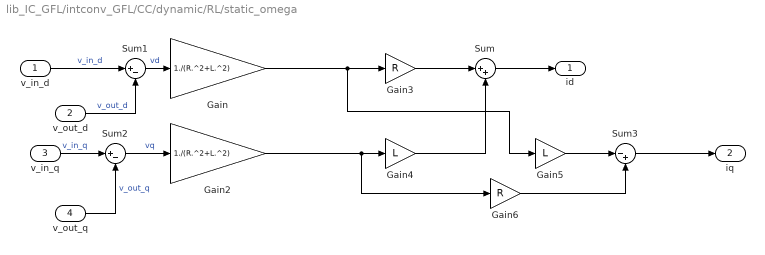
== system lib_IC_GFL/intconv_GFL/CC/dynamic/RL/static_omega ==
  v_in_d : Inport
  v_out_d : Inport  Port=2
  v_in_q : Inport  Port=3
  v_out_q : Inport  Port=4
  Gain : Gain  Gain=1./(R.^2+L.^2)
  Gain2 : Gain  Gain=1./(R.^2+L.^2)
  Gain3 : Gain  Gain=R
  Gain4 : Gain  Gain=L
  Gain5 : Gain  Gain=L
  Gain6 : Gain  Gain=R
  Sum : Sum  Inputs=|++
  Sum1 : Sum  Inputs=|+-
  Sum2 : Sum  Inputs=|+-
  Sum3 : Sum  Inputs=|-+
  id : Outport
  iq : Outport  Port=2
  wires:
  Gain6/1 -> Sum3/2
  Sum3/1 -> iq/1
  Gain5/1 -> Sum3/1
  Sum/1 -> id/1
  Gain2/1 -> Gain4/1, Gain6/1
  Gain4/1 -> Sum/2
  Gain3/1 -> Sum/1
  Gain/1 -> Gain3/1, Gain5/1
  Sum2/1 -> Gain2/1  "vq"
  Sum1/1 -> Gain/1  "vd"
  v_out_d/1 -> Sum1/2  "v_out_d"
  v_out_q/1 -> Sum2/2  "v_out_q"
  v_in_d/1 -> Sum1/1  "v_in_d"
  v_in_q/1 -> Sum2/1  "v_in_q"

== system lib_IC_GFL/intconv_GFL/PC/LPF_d/Active/Impl ==
  In1 : Inport
  Gain : Gain  Gain=iTf
  I : Integrator  InitialCondition=op_intconv_GFL.PC_LPF_d_Active_Impl_I
  Sum4 : Sum  Inputs=|+-
  Out1 : Outport
  wires:
  Gain/1 -> I/1
  Sum4/1 -> Gain/1
  In1/1 -> Sum4/1
  I/1 -> Sum4/2, Out1/1

== system lib_IC_GFL/intconv_GFL/PC/LPF_q/Active/Impl ==
  In1 : Inport
  Gain : Gain  Gain=iTf
  I : Integrator  InitialCondition=op_intconv_GFL.PC_LPF_q_Active_Impl_I
  Sum4 : Sum  Inputs=|+-
  Out1 : Outport
  wires:
  Gain/1 -> I/1
  I/1 -> Sum4/2, Out1/1
  In1/1 -> Sum4/1
  Sum4/1 -> Gain/1
